simulink model "gm_IFFT"  (R2025a)
settings: Solver=VariableStepAuto  StartTime=0.0  StopTime=10.0  RelTol=1e-3
libraries: dsphdlxfrm2 x1
settings Model: Creator=ivanmart  LastModifiedBy=ivanmart
settings OptimizationCC: BlockReduction=off  ConditionallyExecuteInputs=off
settings DebuggingCC: InheritedTsInSrcMsg=none

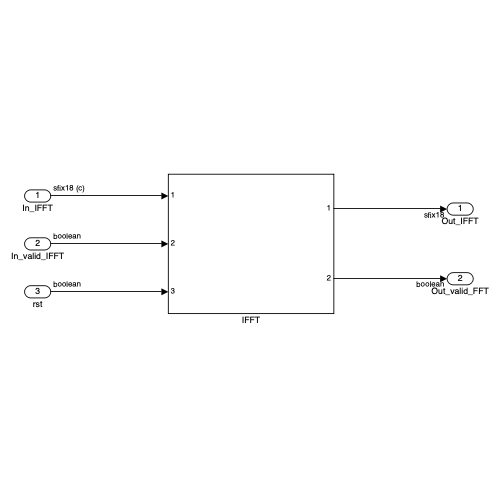
[thumbnail: Simulink's stored preview of the top-level diagram]
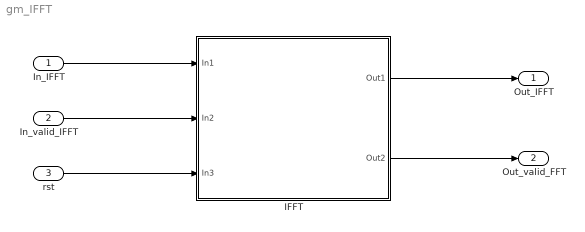
== system gm_IFFT ==
  In_IFFT : Inport  OutDataTypeStr=fixdt(1,18,0)
      settings: SignalType=complex
  In_valid_IFFT : Inport  Port=2  OutDataTypeStr=boolean
  rst : Inport  Port=3  OutDataTypeStr=boolean
  IFFT : Subsystem
  Out_IFFT : Outport  OutDataTypeStr=fixdt(1,18,0)
  Out_valid_FFT : Outport  Port=2  OutDataTypeStr=boolean
  wires:
  IFFT/2(Out2) -> Out_valid_FFT/1
  IFFT/1(Out1) -> Out_IFFT/1
  rst/1 -> IFFT/3(In3)
  In_valid_IFFT/1 -> IFFT/2(In2)
  In_IFFT/1 -> IFFT/1(In1)

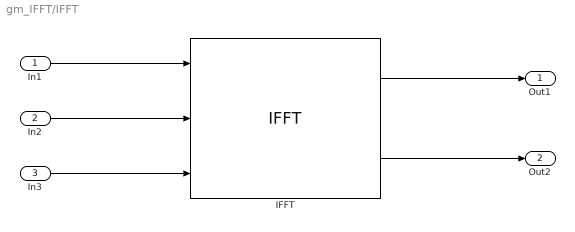
== system gm_IFFT/IFFT ==
  In1 : Inport
  In2 : Inport  Port=2
  In3 : Inport  Port=3
  IFFT : dsphdlxfrm2/IFFT  Architecture=Streaming Radix 2^2  FFTLengthSource=Property  FFTLength=4096  FFTLengthMax=1024  ComplexMultiplication=Use 4 multipliers and 2 adders  BitReversedOutput=off  BitReversedInput=off  Normalize=on  SimulateUsing=Code generation  RoundingMethod=Floor  ResetInputPort=on  StartOutputPort=off  EndOutputPort=off
  Out1 : Outport
  Out2 : Outport  Port=2
  wires:
  In1/1 -> IFFT/1
  In3/1 -> IFFT/3
  In2/1 -> IFFT/2
  IFFT/2 -> Out2/1
  IFFT/1 -> Out1/1
